simulink model "structure_impl_sprayer"  (R2026b)
settings: Solver=VariableStepAuto
undefined symbols (not defined in the file or in its folder): P, Ts
libraries: fl_lib x8, nesl_utility x5, simulink x1
settings Model: Creator=aomar  LastModifiedBy=aomar

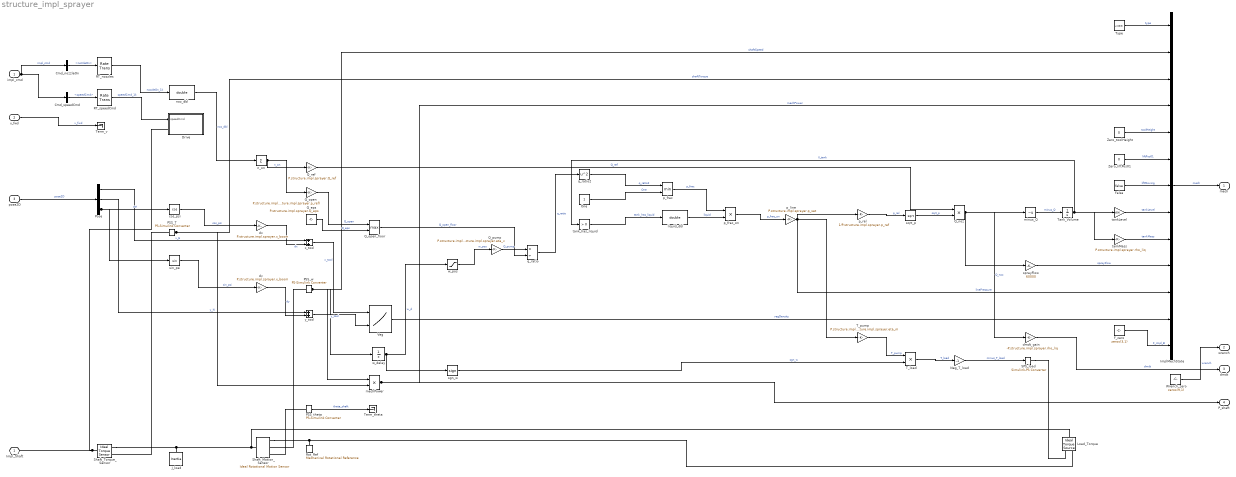
== system structure_impl_sprayer ==
  impl_cmd : Inport  OutDataTypeStr=Bus: Bus_ImplementCmd  SampleTime=Ts.ctrl
  v_fwd : Inport  Port=2
  pose2D : Inport  Port=3
  Cmd_nozzleOn : BusSelector  OutputSignals=nozzleOn
  Cmd_speedCmd : BusSelector  OutputSignals=speedCmd
  Drive : Subsystem  Variant=on
  F_zero : Constant  Value=zeros(3,1)  VectorParams1D=off
  False : Constant  Value=false  VectorParams1D=off  OutDataTypeStr=boolean
  ImplMechState : BusCreator  Inputs=13  OutDataTypeStr=Bus: Bus_ImplMechState  NonVirtualBus=on
  J_load : fl_lib/Mechanical/Rotational Elements/Inertia  inertia=P.structure.impl.sprayer.J kg*m^2  num_ports=foundation.enum.numPorts2.one  w_specify=off  w_priority=High  w=0 rad/s  w_nominal_specify=off  w_nominal_value=1  w_nominal_unit=rad/s  t_specify=off  t_priority=None  t=0 N*m  t_nominal_specify=off  t_nominal_value=1  t_nominal_unit=N*m
  Load_Torque : fl_lib/Mechanical/Mechanical Sources/Ideal Torque Source
  Neg_T_load : Gain  Gain=-1
  One : Constant  VectorParams1D=off
  PSS_T : nesl_utility/PS-Simulink Converter  PhysicalDomain=network_engine_domain  SubClassName=ps_output  LeftPortType=input  RightPortType=output  PseudoPeriodic=off  Frequencies=[]  VectorFormat=inherit  Unit=N*m  AffineConversion=off
  PSS_theta : nesl_utility/PS-Simulink Converter  PhysicalDomain=network_engine_domain  SubClassName=ps_output  LeftPortType=input  RightPortType=output  PseudoPeriodic=off  Frequencies=[]  VectorFormat=inherit  Unit=rad  AffineConversion=off
  PSS_w : nesl_utility/PS-Simulink Converter  PhysicalDomain=network_engine_domain  SubClassName=ps_output  LeftPortType=input  RightPortType=output  PseudoPeriodic=off  Frequencies=[]  VectorFormat=inherit  Unit=rad/s  AffineConversion=off
  Pose : Demux  Outputs=3
  Q_eps : Constant  Value=P.structure.impl.sprayer.Q_eps  VectorParams1D=off
  Q_noz : Product  Inputs=**
  Q_open : Gain  Gain=P.structure.impl.sprayer.Q_ref*sqrt(P.structure.impl.sprayer.p_set/P.structure.impl.sprayer.p_ref)
  Q_open_floor : MinMax  Function=max  Inputs=2  ZeroCross=off
  Q_pump : Gain  Gain=P.structure.impl.sprayer.D_p*P.structure.impl.sprayer.eta_v
  Q_ref : Gain  Gain=P.structure.impl.sprayer.Q_ref
  RT_nozzles : RateTransition  InitialCondition=false(P.structure.impl.sprayer.nNoz,1)  OutPortSampleTime=Ts.base
  RT_speedCmd : RateTransition  OutPortSampleTime=Ts.base
  Rot_Ref : fl_lib/Mechanical/Rotational Elements/Mechanical Rotational Reference
  SPS_load : nesl_utility/Simulink-PS Converter  PhysicalDomain=network_engine_domain  SubClassName=ps_input  LeftPortType=input  RightPortType=output  PseudoPeriodic=off  Frequencies=[]  NoiseDistribution=none  NoiseParameters=[]  Unit=N*m  AffineConversion=off  FilteringAndDerivatives=zero  SimscapeFilterOrder=1  InputFilterTimeConstant=0.001  UdotUserProvided=0
  Shaft_Motion_Sensor : fl_lib/Mechanical/Mechanical Sensors/Ideal Rotational Motion Sensor  reference=foundation.enum.MeasurementReference.difference  acceleration_port=false  velocity_port=true  position_port=true  wrap_angle=false  offset=0 rad
  Shaft_Torque_Sensor : fl_lib/Mechanical/Mechanical Sensors/Ideal Torque Sensor
  T_load : Product  Inputs=**
  T_pump : Gain  Gain=P.structure.impl.sprayer.D_p/P.structure.impl.sprayer.eta_m
  Tank_Volume : Integrator  InitialCondition=P.structure.impl.sprayer.fill0*P.structure.impl.sprayer.V_max  LimitOutput=on  UpperSaturationLimit=P.structure.impl.sprayer.V_max  LowerSaturationLimit=0  ZeroCross=off
  Term_theta : Terminator
  Term_v : Terminator
  Type : Constant  Value=uint8(3)  VectorParams1D=off  OutDataTypeStr=uint8
  Veg : Lookup_n-D  BreakpointsForDimension1=P.world.terrain.xE  BreakpointsForDimension2=P.world.terrain.yN  IndexSearchMethod=Evenly spaced points  Table=P.world.veg.rho  ExtrapMethod=Clip  InternalRulePriority=Speed  RndMeth=Simplest
      settings: InputPortMap=u0,u1
  Wrench_zero : Constant  Value=zeros(9,1)  VectorParams1D=off
  Zero_liftPos01 : Constant  Value=0  VectorParams1D=off
  Zero_toolHeight : Constant  Value=0  VectorParams1D=off
  cos_psi : Trigonometry  Operator=cos
  dmdt_gain : Gain  Gain=-P.structure.impl.sprayer.rho_liq
  dx : Gain  Gain=P.structure.impl.sprayer.x_boom
  dy : Gain  Gain=P.structure.impl.sprayer.x_boom
  liquid_dbl : DataTypeConversion  OutDataTypeStr=double  SaturateOnIntegerOverflow=off  RndMeth=Floor
  mechPower : Product  Inputs=**
  minus_Q : UnaryMinus
  n_on : Sum  Inputs=+
  noz_dbl : DataTypeConversion  OutDataTypeStr=double  SaturateOnIntegerOverflow=off  RndMeth=Floor
  p_frac : MinMax  Inputs=2  ZeroCross=off
  p_frac_on : Product  Inputs=**
  p_line : Gain  Gain=P.structure.impl.sprayer.p_set
  p_rel : Gain  Gain=1/P.structure.impl.sprayer.p_ref
  q_ratio : Product  Inputs=*/
  q_ratio2 : Math  Operator=square
  sgn_w : Signum  ZeroCross=off
  sin_psi : Trigonometry
  sprayFlow : Gain  Gain=60000
  sqrt_p : Sqrt
  tankLevel : Gain  Gain=1000
  tankMass : Gain  Gain=P.structure.impl.sprayer.rho_liq
  tank_has_liquid : simulink/Logic and Bit Operations/Compare To Zero  relop=>  OutDataTypeStr=boolean
  w_delay : UnitDelay  SampleTime=Ts.base
  w_pos : Saturate  UpperLimit=inf  LowerLimit=0
  x_tool : Sum
  y_tool : Sum
  Impl_Shaft : PMIOPort  Side=Left  ConnectionType=Connection: foundation.mechanical.rotational.rotational
  mech : Outport  OutDataTypeStr=Bus: Bus_ImplMechState
  wrench : Outport  Port=2
  dmdt : Outport  Port=3
  P_shaft : Outport  Port=4
  wires:
  impl_cmd/1 -> Cmd_speedCmd/1, Cmd_nozzleOn/1  "impl_cmd"
  v_fwd/1 -> Term_v/1  "v_fwd"
  pose2D/1 -> Pose/1  "pose2D"
  Cmd_nozzleOn/1 -> RT_nozzles/1  "<nozzleOn>"
  Cmd_speedCmd/1 -> RT_speedCmd/1  "<speedCmd>"
  Pose/1 -> x_tool/1  "x_E"
  Pose/2 -> y_tool/1  "y_N"
  Pose/3 -> sin_psi/1, cos_psi/1  "psi"
  RT_nozzles/1 -> noz_dbl/1  "nozzleOn_1k"
  RT_speedCmd/1 -> Drive/1(speedCmd)  "speedCmd_1k"
  PSS_T/1 -> mechPower/2, ImplMechState/3  "shaftTorque"
  cos_psi/1 -> dx/1  "cos_psi"
  sin_psi/1 -> dy/1  "sin_psi"
  noz_dbl/1 -> n_on/1  "noz_dbl"
  n_on/1 -> Q_open/1, Q_ref/1  "n_on"
  dx/1 -> x_tool/2  "dx"
  dy/1 -> y_tool/2  "dy"
  PSS_w/1 -> ImplMechState/2, mechPower/1, w_delay/1  "shaftSpeed"
  PSS_theta/1 -> Term_theta/1  "theta_shaft"
  x_tool/1 -> Veg/1  "x_tool"
  y_tool/1 -> Veg/2  "y_tool"
  Q_ref/1 -> Q_noz/1  "Q_ref"
  Q_open/1 -> Q_open_floor/1  "Q_open"
  Q_eps/1 -> Q_open_floor/2  "Q_eps"
  Q_open_floor/1 -> q_ratio/2  "Q_open_floor"
  mechPower/1 -> ImplMechState/4, P_shaft/1  "mechPower"
  w_delay/1 -> w_pos/1, sgn_w/1  "w_d"
  Veg/1 -> ImplMechState/12  "vegDensity"
  w_pos/1 -> Q_pump/1  "w_pos"
  sgn_w/1 -> T_load/2  "sgn_w"
  Q_pump/1 -> q_ratio/1  "Q_pump"
  q_ratio/1 -> q_ratio2/1  "q_ratio"
  q_ratio2/1 -> p_frac/1  "q_ratio2"
  One/1 -> p_frac/2  "One"
  tank_has_liquid/1 -> liquid_dbl/1  "tank_has_liquid"
  p_frac/1 -> p_frac_on/1  "p_frac"
  liquid_dbl/1 -> p_frac_on/2  "liquid"
  p_frac_on/1 -> p_line/1  "p_frac_on"
  p_line/1 -> T_pump/1, ImplMechState/11, p_rel/1  "linePressure"
  p_rel/1 -> sqrt_p/1  "p_rel"
  T_pump/1 -> T_load/1  "T_pump"
  sqrt_p/1 -> Q_noz/2  "sqrt_p"
  T_load/1 -> Neg_T_load/1  "T_load"
  Q_noz/1 -> dmdt_gain/1, sprayFlow/1, minus_Q/1  "Q_noz"
  Neg_T_load/1 -> SPS_load/1  "minus_T_load"
  minus_Q/1 -> Tank_Volume/1  "minus_Q"
  sprayFlow/1 -> ImplMechState/10  "sprayFlow"
  dmdt_gain/1 -> dmdt/1  "dmdt"
  Tank_Volume/1 -> tankMass/1, tank_has_liquid/1, tankLevel/1  "V_tank"
  Type/1 -> ImplMechState/1  "type"
  Zero_toolHeight/1 -> ImplMechState/5  "toolHeight"
  Zero_liftPos01/1 -> ImplMechState/6  "liftPos01"
  False/1 -> ImplMechState/7  "liftMoving"
  tankLevel/1 -> ImplMechState/8  "tankLevel"
  tankMass/1 -> ImplMechState/9  "tankMass"
  F_zero/1 -> ImplMechState/13  "F_impl_B"
  ImplMechState/1 -> mech/1  "mech"
  Wrench_zero/1 -> wrench/1  "wrench"
  connections:
  Shaft_Torque_Sensor/LConn1 -- Drive/LConn1 -- Impl_Shaft/RConn1
  J_load/LConn1 -- Shaft_Torque_Sensor/RConn1 -- Shaft_Motion_Sensor/LConn1 -- Load_Torque/LConn1
  SPS_load/RConn1 -- Load_Torque/RConn1
  Rot_Ref/LConn1 -- Shaft_Motion_Sensor/RConn1 -- Load_Torque/RConn2
  PSS_T/LConn1 -- Shaft_Torque_Sensor/RConn2
  PSS_theta/LConn1 -- Shaft_Motion_Sensor/RConn3
  PSS_w/LConn1 -- Shaft_Motion_Sensor/RConn2

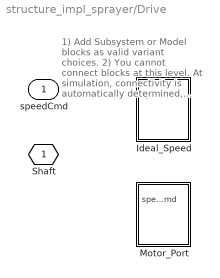
== system structure_impl_sprayer/Drive ==
  note: 1) Add Subsystem or Model blocks as valid variant choices.
      | 2) You cannot connect blocks at this level. At simulation, connectivity is automatically
      | determined, based on the active variant and port name matching.
  speedCmd : Inport
  Ideal_Speed : Subsystem  VariantControl=VC_IMPL_DRIVE == 1
  Motor_Port : Subsystem  VariantControl=VC_IMPL_DRIVE == 2
  Shaft : PMIOPort  Side=Left  ConnectionType=Connection: foundation.mechanical.rotational.rotational

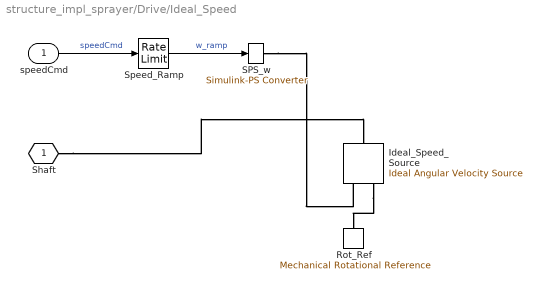
== system structure_impl_sprayer/Drive/Ideal_Speed ==
  speedCmd : Inport
  Ideal_Speed_Source : fl_lib/Mechanical/Mechanical Sources/Ideal Angular Velocity Source
  Rot_Ref : fl_lib/Mechanical/Rotational Elements/Mechanical Rotational Reference
  SPS_w : nesl_utility/Simulink-PS Converter  PhysicalDomain=network_engine_domain  SubClassName=ps_input  LeftPortType=input  RightPortType=output  PseudoPeriodic=off  Frequencies=[]  NoiseDistribution=none  NoiseParameters=[]  Unit=rad/s  AffineConversion=off  FilteringAndDerivatives=filter  SimscapeFilterOrder=1  InputFilterTimeConstant=P.structure.impl.drive.tau_f  UdotUserProvided=0
  Speed_Ramp : RateLimiter  RisingSlewLimit=P.structure.impl.drive.a_max  FallingSlewLimit=-P.structure.impl.drive.a_max  SampleTimeMode=inherited
  Shaft : PMIOPort  Side=Left  ConnectionType=Connection: foundation.mechanical.rotational.rotational
  wires:
  speedCmd/1 -> Speed_Ramp/1  "speedCmd"
  Speed_Ramp/1 -> SPS_w/1  "w_ramp"
  connections:
  Shaft/RConn1 -- Ideal_Speed_Source/LConn1
  SPS_w/RConn1 -- Ideal_Speed_Source/RConn1
  Ideal_Speed_Source/RConn2 -- Rot_Ref/LConn1

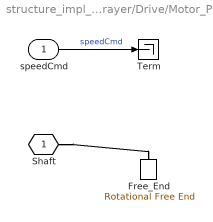
== system structure_impl_sprayer/Drive/Motor_Port ==
  speedCmd : Inport
  Free_End : fl_lib/Mechanical/Rotational Elements/Rotational Free End  w_specify=off  w_priority=None  w=0 rad/s  w_nominal_specify=off  w_nominal_value=1  w_nominal_unit=rad/s
  Term : Terminator
  Shaft : PMIOPort  Side=Left  ConnectionType=Connection: foundation.mechanical.rotational.rotational
  wires:
  speedCmd/1 -> Term/1  "speedCmd"
  connections:
  Shaft/RConn1 -- Free_End/LConn1
